simulink model "generic_src"  (Simulink 10.3)
settings: Solver=ode45  StartTime=0.0  StopTime=inf  RelTol=1e-3  EnableMultiTasking=on
undefined symbols (not defined in the file or in its folder): Area_Front, Area_Rear, ay_max_off, ay_max_on, ay_per_mu_max_off, ay_per_mu_max_on, Brake_ratio, brake_valve_ctrl_kP, cat1mode1_higher, cat1mode1_lower, cat1mode2_higher, cat1mode2_lower, cat1mode3_higher, cat1mode3_lower, cat2mode1_higher, cat2mode1_lower, cat2mode2_higher, cat2mode2_lower, cat2mode3_higher, cat2mode3_lower, delta_vel, diff_lock_fac, diff_lock_off, diff_lock_on, ESP_ctrl_kD, ESP_ctrl_kI, ESP_ctrl_kP, ESP_ctrl_restore_kI, ESP_min_throttle_fac, f_ax, f_slip, g, higherlimit_highvel, higherlimit_lowvel, highervel_fac, highervelocity_fac, InitialConditionForIntegrator, limit_acc, limit_selectlow, limit_starting, limit_vdiff, locktime_throttle, lowerlimit_highvel, lowerlimit_lowvel, lowervel_fac, lowervelocity_fac, min_throttle, MPS2KMPH, MSR_ctrl_kD, MSR_ctrl_kI, MSR_ctrl_kP, MSR_min_throttle_fac, PID_kP_sideslip, PID_kP_yawrate, RADpS2RpM, rBrake, RpM2RADpS, SH_SL_switch, sideslip_vel_corr, sidesplip_deviation_max ... (+35)
libraries: CarMaker4SL x136, simulink x55, simulink_extras x6
(part 3 of 9)

== system generic_src/CarMaker/IPG Vehicle/PowerTrain/PTControl Example/PTC MotorOut ==
  BusCreator : BusCreator  Inputs=12
  CreateBus PTC MotorOut0 : Subsystem
  CreateBus PTC MotorOut1 : Subsystem
  CreateBus PTC MotorOut10 : Subsystem
  CreateBus PTC MotorOut11 : Subsystem
  CreateBus PTC MotorOut2 : Subsystem
  CreateBus PTC MotorOut3 : Subsystem
  CreateBus PTC MotorOut4 : Subsystem
  CreateBus PTC MotorOut5 : Subsystem
  CreateBus PTC MotorOut6 : Subsystem
  CreateBus PTC MotorOut7 : Subsystem
  CreateBus PTC MotorOut8 : Subsystem
  CreateBus PTC MotorOut9 : Subsystem
  Ground PTC MotorOut{0..11} (12 alike) : Ground
  PTC MotorOut : Outport
  wires:
  CreateBus PTC MotorOut0/1(Out) -> BusCreator/1  "PTC MotorOut0"
  Ground PTC MotorOut0/1 -> CreateBus PTC MotorOut0/1(In)
  Ground PTC MotorOut3/1 -> CreateBus PTC MotorOut3/1(In)
  Ground PTC MotorOut1/1 -> CreateBus PTC MotorOut1/1(In)
  CreateBus PTC MotorOut1/1(Out) -> BusCreator/2  "PTC MotorOut1"
  Ground PTC MotorOut4/1 -> CreateBus PTC MotorOut4/1(In)
  Ground PTC MotorOut2/1 -> CreateBus PTC MotorOut2/1(In)
  CreateBus PTC MotorOut2/1(Out) -> BusCreator/3  "PTC MotorOut2"
  Ground PTC MotorOut5/1 -> CreateBus PTC MotorOut5/1(In)
  Ground PTC MotorOut6/1 -> CreateBus PTC MotorOut6/1(In)
  Ground PTC MotorOut7/1 -> CreateBus PTC MotorOut7/1(In)
  Ground PTC MotorOut8/1 -> CreateBus PTC MotorOut8/1(In)
  Ground PTC MotorOut9/1 -> CreateBus PTC MotorOut9/1(In)
  Ground PTC MotorOut10/1 -> CreateBus PTC MotorOut10/1(In)
  Ground PTC MotorOut11/1 -> CreateBus PTC MotorOut11/1(In)
  CreateBus PTC MotorOut4/1(Out) -> BusCreator/5  "PTC MotorOut4"
  CreateBus PTC MotorOut5/1(Out) -> BusCreator/6  "PTC MotorOut5"
  CreateBus PTC MotorOut6/1(Out) -> BusCreator/7  "PTC MotorOut6"
  CreateBus PTC MotorOut7/1(Out) -> BusCreator/8  "PTC MotorOut7"
  CreateBus PTC MotorOut8/1(Out) -> BusCreator/9  "PTC MotorOut8"
  CreateBus PTC MotorOut9/1(Out) -> BusCreator/10  "PTC MotorOut9"
  CreateBus PTC MotorOut10/1(Out) -> BusCreator/11  "PTC MotorOut10"
  CreateBus PTC MotorOut11/1(Out) -> BusCreator/12  "PTC MotorOut11"
  CreateBus PTC MotorOut3/1(Out) -> BusCreator/4  "PTC MotorOut3"
  BusCreator/1 -> PTC MotorOut/1  "CreateBus PTC MotorOut"

== system generic_src/CarMaker/IPG Vehicle/PowerTrain/PTControl Example/PTControl Example ==
  note: Minimalistic PTControl example model, that only works with
      | the 'Generic' powertrain and the 'Manual' gearbox.
  EngineIn : Inport
  VhclCtrl.PT : Inport  Port=2
  Bus Selector : BusSelector  OutputSignals=VhclCtrl Key,VhclCtrl Gas,VhclCtrl Clutch,VhclCtrl GearNo
  Bus Selector1 : BusSelector  OutputSignals=PTC EngineIn.PTC EngineIn Engine_on
  Engine : Subsystem
  ISG : Subsystem
  PTC : Subsystem
  PTC MiscOut : Outport  VectorParamsAs1DForOutWhenUnconnected=off
  EngineOut : Outport  Port=2  VectorParamsAs1DForOutWhenUnconnected=off
  ISGOut : Outport  Port=3  VectorParamsAs1DForOutWhenUnconnected=off
  ClutchOut Pos : Outport  Port=4  VectorParamsAs1DForOutWhenUnconnected=off
  GearBoxOut GearNoTrg : Outport  Port=5  VectorParamsAs1DForOutWhenUnconnected=off
  wires:
  VhclCtrl.PT/1 -> Bus Selector/1
  EngineIn/1 -> Bus Selector1/1
  Engine/1(EngineOut) -> EngineOut/1
  Bus Selector1/1 -> Engine/2(Engine_on), PTC/2(Engine_on)  "<PTC EngineIn Engine_on>"
  Bus Selector/2 -> Engine/1(Gas)  "<VhclCtrl Gas>"
  ISG/1(ISGOut) -> ISGOut/1
  PTC/1(PTC MiscOut) -> PTC MiscOut/1
  Bus Selector/4 -> GearBoxOut GearNoTrg/1  "<VhclCtrl GearNo>"
  Bus Selector/3 -> ClutchOut Pos/1  "<VhclCtrl Clutch>"
  Bus Selector/1 -> PTC/1(Key), ISG/1(Key)  "<VhclCtrl Key>"

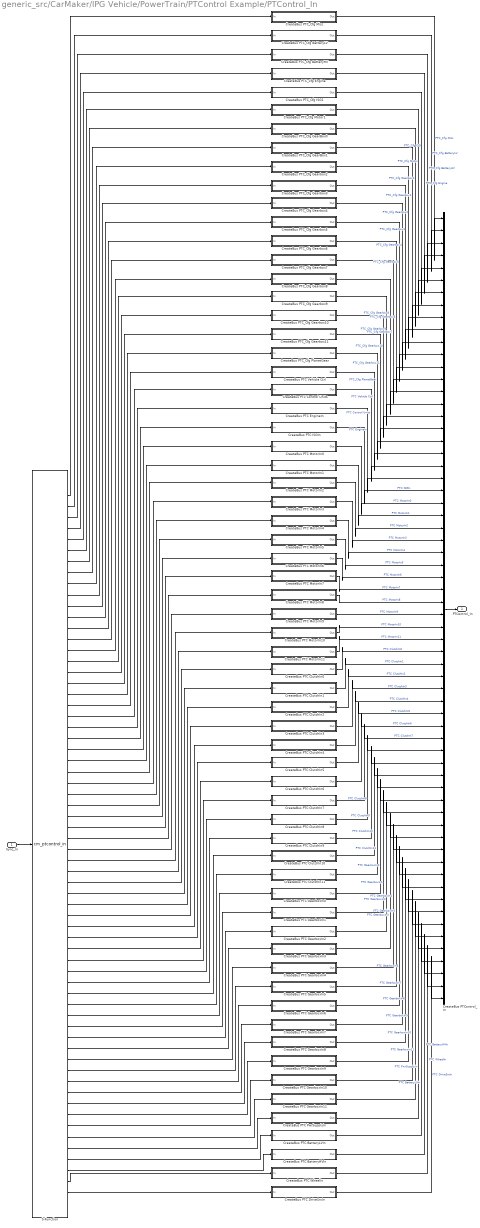
== system generic_src/CarMaker/IPG Vehicle/PowerTrain/PTControl Example/PTControl_In ==
  Sync_In : Inport
  CreateBus PTC BatteryHVIn : Subsystem
  CreateBus PTC BatteryLVIn : Subsystem
  CreateBus PTC ClutchIn0 : Subsystem
  CreateBus PTC ClutchIn1 : Subsystem
  CreateBus PTC ClutchIn10 : Subsystem
  CreateBus PTC ClutchIn11 : Subsystem
  CreateBus PTC ClutchIn2 : Subsystem
  CreateBus PTC ClutchIn3 : Subsystem
  CreateBus PTC ClutchIn4 : Subsystem
  CreateBus PTC ClutchIn5 : Subsystem
  CreateBus PTC ClutchIn6 : Subsystem
  CreateBus PTC ClutchIn7 : Subsystem
  CreateBus PTC ClutchIn8 : Subsystem
  CreateBus PTC ClutchIn9 : Subsystem
  CreateBus PTC Control Units : Subsystem
  CreateBus PTC DriveSrcIn : Subsystem
  CreateBus PTC EngineIn : Subsystem
  CreateBus PTC GearboxIn0 : Subsystem
  CreateBus PTC GearboxIn1 : Subsystem
  CreateBus PTC GearboxIn10 : Subsystem
  CreateBus PTC GearboxIn11 : Subsystem
  CreateBus PTC GearboxIn2 : Subsystem
  CreateBus PTC GearboxIn3 : Subsystem
  CreateBus PTC GearboxIn4 : Subsystem
  CreateBus PTC GearboxIn5 : Subsystem
  CreateBus PTC GearboxIn6 : Subsystem
  CreateBus PTC GearboxIn7 : Subsystem
  CreateBus PTC GearboxIn8 : Subsystem
  CreateBus PTC GearboxIn9 : Subsystem
  CreateBus PTC ISGIn : Subsystem
  CreateBus PTC MotorIn0 : Subsystem
  CreateBus PTC MotorIn1 : Subsystem
  CreateBus PTC MotorIn10 : Subsystem
  CreateBus PTC MotorIn11 : Subsystem
  CreateBus PTC MotorIn2 : Subsystem
  CreateBus PTC MotorIn3 : Subsystem
  CreateBus PTC MotorIn4 : Subsystem
  CreateBus PTC MotorIn5 : Subsystem
  CreateBus PTC MotorIn6 : Subsystem
  CreateBus PTC MotorIn7 : Subsystem
  CreateBus PTC MotorIn8 : Subsystem
  CreateBus PTC MotorIn9 : Subsystem
  CreateBus PTC PwrSupplyIn : Subsystem
  CreateBus PTC Vehicle Ctrl : Subsystem
  CreateBus PTC WheelIn : Subsystem
  CreateBus PTC_Cfg BatteryHV : Subsystem
  CreateBus PTC_Cfg BatteryLV : Subsystem
  CreateBus PTC_Cfg Engine : Subsystem
  CreateBus PTC_Cfg GearBox0 : Subsystem
  CreateBus PTC_Cfg GearBox1 : Subsystem
  CreateBus PTC_Cfg Gearbox10 : Subsystem
  CreateBus PTC_Cfg Gearbox11 : Subsystem
  CreateBus PTC_Cfg Gearbox2 : Subsystem
  CreateBus PTC_Cfg Gearbox3 : Subsystem
  CreateBus PTC_Cfg Gearbox4 : Subsystem
  CreateBus PTC_Cfg Gearbox5 : Subsystem
  CreateBus PTC_Cfg Gearbox6 : Subsystem
  CreateBus PTC_Cfg Gearbox7 : Subsystem
  CreateBus PTC_Cfg Gearbox8 : Subsystem
  CreateBus PTC_Cfg Gearbox9 : Subsystem
  CreateBus PTC_Cfg ISG1 : Subsystem
  CreateBus PTC_Cfg Misc : Subsystem
  CreateBus PTC_Cfg Motor1 : Subsystem
  CreateBus PTC_Cfg PlanetGear : Subsystem
  CreateBus PTControl_In : BusCreator  Inputs=64
  S-Function : S-Function  FunctionName=cm_ptcontrol_in  SFunctionDeploymentMode=off  EnableBusSupport=off
  PTControl_In : Outport  VectorParamsAs1DForOutWhenUnconnected=off
  wires:
  CreateBus PTControl_In/1 -> PTControl_In/1
  Sync_In/1 -> S-Function/1
  S-Function/2 -> CreateBus PTC_Cfg BatteryLV/1(In)
  CreateBus PTC_Cfg Misc/1(Out) -> CreateBus PTControl_In/1  "PTC_Cfg Misc"
  S-Function/1 -> CreateBus PTC_Cfg Misc/1(In)
  CreateBus PTC_Cfg Motor1/1(Out) -> CreateBus PTControl_In/6  "PTC_Cfg Motor"
  CreateBus PTC_Cfg Gearbox2/1(Out) -> CreateBus PTControl_In/9  "PTC_Cfg Gearbox2"
  S-Function/4 -> CreateBus PTC_Cfg Engine/1(In)
  S-Function/3 -> CreateBus PTC_Cfg BatteryHV/1(In)
  S-Function/7 -> CreateBus PTC_Cfg GearBox0/1(In)
  S-Function/14 -> CreateBus PTC_Cfg Gearbox7/1(In)
  S-Function/15 -> CreateBus PTC_Cfg Gearbox8/1(In)
  S-Function/17 -> CreateBus PTC_Cfg Gearbox10/1(In)
  S-Function/18 -> CreateBus PTC_Cfg Gearbox11/1(In)
  CreateBus PTC_Cfg GearBox1/1(Out) -> CreateBus PTControl_In/8  "PTC_Cfg Gearbox1"
  CreateBus PTC_Cfg Gearbox4/1(Out) -> CreateBus PTControl_In/11  "PTC_Cfg Gearbox4"
  CreateBus PTC_Cfg Gearbox5/1(Out) -> CreateBus PTControl_In/12  "PTC_Cfg Gearbox5"
  CreateBus PTC_Cfg Gearbox6/1(Out) -> CreateBus PTControl_In/13  "PTC_Cfg Gearbox6"
  CreateBus PTC_Cfg Gearbox7/1(Out) -> CreateBus PTControl_In/14  "PTC_Cfg Gearbox7"
  CreateBus PTC GearboxIn6/1(Out) -> CreateBus PTControl_In/54  "PTC GearboxIn6"
  CreateBus PTC ClutchIn6/1(Out) -> CreateBus PTControl_In/42  "PTC ClutchIn6"
  CreateBus PTC GearboxIn5/1(Out) -> CreateBus PTControl_In/53  "PTC GearboxIn5"
  CreateBus PTC GearboxIn9/1(Out) -> CreateBus PTControl_In/57  "PTC GearboxIn9"
  CreateBus PTC ClutchIn8/1(Out) -> CreateBus PTControl_In/44  "PTC ClutchIn8"
  S-Function/32 -> CreateBus PTC MotorIn8/1(In)
  CreateBus PTC MotorIn0/1(Out) -> CreateBus PTControl_In/24  "PTC MotorIn0"
  S-Function/8 -> CreateBus PTC_Cfg GearBox1/1(In)
  S-Function/46 -> CreateBus PTC ClutchIn10/1(In)
  S-Function/61 -> CreateBus PTC BatteryLVIn/1(In)
  S-Function/11 -> CreateBus PTC_Cfg Gearbox4/1(In)
  S-Function/37 -> CreateBus PTC ClutchIn1/1(In)
  S-Function/50 -> CreateBus PTC GearboxIn2/1(In)
  CreateBus PTC WheelIn/1(Out) -> CreateBus PTControl_In/63  "PTC WheelIn"
  S-Function/24 -> CreateBus PTC MotorIn0/1(In)
  CreateBus PTC_Cfg Gearbox3/1(Out) -> CreateBus PTControl_In/10  "PTC_Cfg Gearbox3"
  S-Function/51 -> CreateBus PTC GearboxIn3/1(In)
  S-Function/56 -> CreateBus PTC GearboxIn8/1(In)
  CreateBus PTC GearboxIn3/1(Out) -> CreateBus PTControl_In/51  "PTC GearboxIn3"
  CreateBus PTC MotorIn1/1(Out) -> CreateBus PTControl_In/25  "PTC MotorIn1"
  S-Function/10 -> CreateBus PTC_Cfg Gearbox3/1(In)
  CreateBus PTC DriveSrcIn/1(Out) -> CreateBus PTControl_In/64  "PTC DriveSrcIn"
  CreateBus PTC ISGIn/1(Out) -> CreateBus PTControl_In/23  "PTC ISGIn"
  CreateBus PTC ClutchIn11/1(Out) -> CreateBus PTControl_In/47  "PTC ClutchIn11"
  S-Function/20 -> CreateBus PTC Vehicle Ctrl/1(In)
  S-Function/47 -> CreateBus PTC ClutchIn11/1(In)
  S-Function/64 -> CreateBus PTC DriveSrcIn/1(In)
  CreateBus PTC ClutchIn10/1(Out) -> CreateBus PTControl_In/46  "PTC ClutchIn10"
  CreateBus PTC GearboxIn2/1(Out) -> CreateBus PTControl_In/50  "PTC GearboxIn2"
  CreateBus PTC GearboxIn0/1(Out) -> CreateBus PTControl_In/48  "PTC GearboxIn0"
  S-Function/16 -> CreateBus PTC_Cfg Gearbox9/1(In)
  S-Function/25 -> CreateBus PTC MotorIn1/1(In)
  S-Function/63 -> CreateBus PTC WheelIn/1(In)
  CreateBus PTC GearboxIn1/1(Out) -> CreateBus PTControl_In/49  "PTC GearboxIn1"
  S-Function/33 -> CreateBus PTC MotorIn9/1(In)
  CreateBus PTC BatteryLVIn/1(Out) -> CreateBus PTControl_In/61  "PTC BatteryLVIn"
  S-Function/58 -> CreateBus PTC GearboxIn10/1(In)
  S-Function/41 -> CreateBus PTC ClutchIn5/1(In)
  S-Function/5 -> CreateBus PTC_Cfg ISG1/1(In)
  S-Function/44 -> CreateBus PTC ClutchIn8/1(In)
  S-Function/45 -> CreateBus PTC ClutchIn9/1(In)
  CreateBus PTC GearboxIn11/1(Out) -> CreateBus PTControl_In/59  "PTC GearboxIn11"
  S-Function/9 -> CreateBus PTC_Cfg Gearbox2/1(In)
  S-Function/35 -> CreateBus PTC MotorIn11/1(In)
  S-Function/19 -> CreateBus PTC_Cfg PlanetGear/1(In)
  CreateBus PTC GearboxIn8/1(Out) -> CreateBus PTControl_In/56  "PTC GearboxIn8"
  S-Function/36 -> CreateBus PTC ClutchIn0/1(In)
  S-Function/53 -> CreateBus PTC GearboxIn5/1(In)
  CreateBus PTC GearboxIn10/1(Out) -> CreateBus PTControl_In/58  "PTC GearboxIn10"
  S-Function/6 -> CreateBus PTC_Cfg Motor1/1(In)
  CreateBus PTC PwrSupplyIn/1(Out) -> CreateBus PTControl_In/60  "PTC PwrSupplyIn"
  S-Function/43 -> CreateBus PTC ClutchIn7/1(In)
  CreateBus PTC_Cfg BatteryLV/1(Out) -> CreateBus PTControl_In/2  "PTC_Cfg BatteryLV"
  CreateBus PTC ClutchIn1/1(Out) -> CreateBus PTControl_In/37  "PTC ClutchIn1"
  S-Function/26 -> CreateBus PTC MotorIn2/1(In)
  CreateBus PTC_Cfg PlanetGear/1(Out) -> CreateBus PTControl_In/19  "PTC_Cfg PlanetGear"
  CreateBus PTC_Cfg Gearbox10/1(Out) -> CreateBus PTControl_In/17  "PTC_Cfg Gearbox10"
  CreateBus PTC ClutchIn7/1(Out) -> CreateBus PTControl_In/43  "PTC ClutchIn7"
  S-Function/54 -> CreateBus PTC GearboxIn6/1(In)
  S-Function/29 -> CreateBus PTC MotorIn5/1(In)
  CreateBus PTC_Cfg BatteryHV/1(Out) -> CreateBus PTControl_In/3  "PTC_Cfg BatteryHV"
  S-Function/13 -> CreateBus PTC_Cfg Gearbox6/1(In)
  CreateBus PTC ClutchIn9/1(Out) -> CreateBus PTControl_In/45  "PTC ClutchIn9"
  CreateBus PTC GearboxIn4/1(Out) -> CreateBus PTControl_In/52  "PTC GearboxIn4"
  S-Function/57 -> CreateBus PTC GearboxIn9/1(In)
  CreateBus PTC GearboxIn7/1(Out) -> CreateBus PTControl_In/55  "PTC GearboxIn7"
  S-Function/60 -> CreateBus PTC PwrSupplyIn/1(In)
  CreateBus PTC BatteryHVIn/1(Out) -> CreateBus PTControl_In/62  "PTC BatteryHVIn"
  S-Function/49 -> CreateBus PTC GearboxIn1/1(In)
  S-Function/55 -> CreateBus PTC GearboxIn7/1(In)
  S-Function/21 -> CreateBus PTC Control Units/1(In)
  CreateBus PTC ClutchIn5/1(Out) -> CreateBus PTControl_In/41  "PTC ClutchIn5"
  CreateBus PTC ClutchIn4/1(Out) -> CreateBus PTControl_In/40  "PTC ClutchIn4"
  S-Function/38 -> CreateBus PTC ClutchIn2/1(In)
  CreateBus PTC Control Units/1(Out) -> CreateBus PTControl_In/21  "PTC Control Units"
  S-Function/40 -> CreateBus PTC ClutchIn4/1(In)
  CreateBus PTC MotorIn11/1(Out) -> CreateBus PTControl_In/35  "PTC MotorIn11"
  CreateBus PTC ClutchIn3/1(Out) -> CreateBus PTControl_In/39  "PTC ClutchIn3"
  S-Function/39 -> CreateBus PTC ClutchIn3/1(In)
  CreateBus PTC MotorIn2/1(Out) -> CreateBus PTControl_In/26  "PTC MotorIn2"
  CreateBus PTC ClutchIn2/1(Out) -> CreateBus PTControl_In/38  "PTC ClutchIn2"
  CreateBus PTC_Cfg ISG1/1(Out) -> CreateBus PTControl_In/5  "PTC_Cfg ISG"
  CreateBus PTC ClutchIn0/1(Out) -> CreateBus PTControl_In/36  "PTC ClutchIn0"
  S-Function/52 -> CreateBus PTC GearboxIn4/1(In)
  CreateBus PTC EngineIn/1(Out) -> CreateBus PTControl_In/22  "PTC EngineIn"
  CreateBus PTC_Cfg GearBox0/1(Out) -> CreateBus PTControl_In/7  "PTC_Cfg Gearbox0"
  S-Function/42 -> CreateBus PTC ClutchIn6/1(In)
  S-Function/34 -> CreateBus PTC MotorIn10/1(In)
  CreateBus PTC MotorIn9/1(Out) -> CreateBus PTControl_In/33  "PTC MotorIn9"
  S-Function/30 -> CreateBus PTC MotorIn6/1(In)
  S-Function/12 -> CreateBus PTC_Cfg Gearbox5/1(In)
  CreateBus PTC MotorIn8/1(Out) -> CreateBus PTControl_In/32  "PTC MotorIn8"
  CreateBus PTC MotorIn7/1(Out) -> CreateBus PTControl_In/31  "PTC MotorIn7"
  S-Function/31 -> CreateBus PTC MotorIn7/1(In)
  CreateBus PTC MotorIn6/1(Out) -> CreateBus PTControl_In/30  "PTC MotorIn6"
  CreateBus PTC MotorIn4/1(Out) -> CreateBus PTControl_In/28  "PTC MotorIn4"
  S-Function/62 -> CreateBus PTC BatteryHVIn/1(In)
  S-Function/27 -> CreateBus PTC MotorIn3/1(In)
  S-Function/28 -> CreateBus PTC MotorIn4/1(In)
  CreateBus PTC MotorIn5/1(Out) -> CreateBus PTControl_In/29  "PTC MotorIn5"
  CreateBus PTC MotorIn3/1(Out) -> CreateBus PTControl_In/27  "PTC MotorIn3"
  S-Function/23 -> CreateBus PTC ISGIn/1(In)
  S-Function/22 -> CreateBus PTC EngineIn/1(In)
  CreateBus PTC_Cfg Engine/1(Out) -> CreateBus PTControl_In/4  "PTC_Cfg Engine"
  S-Function/48 -> CreateBus PTC GearboxIn0/1(In)
  S-Function/59 -> CreateBus PTC GearboxIn11/1(In)
  CreateBus PTC Vehicle Ctrl/1(Out) -> CreateBus PTControl_In/20  "PTC Vehicle Ctrl"
  CreateBus PTC MotorIn10/1(Out) -> CreateBus PTControl_In/34  "PTC MotorIn10"
  CreateBus PTC_Cfg Gearbox11/1(Out) -> CreateBus PTControl_In/18  "PTC_Cfg Gearbox11"
  CreateBus PTC_Cfg Gearbox9/1(Out) -> CreateBus PTControl_In/16  "PTC_Cfg Gearbox9"
  CreateBus PTC_Cfg Gearbox8/1(Out) -> CreateBus PTControl_In/15  "PTC_Cfg Gearbox8"

== system generic_src/CarMaker/IPG Vehicle/PowerTrain/PTControl Example/PTControl_Out ==
  PTC MiscOut : Inport
  PTC EngineOut : Inport  Port=2
  PTC ISGOut : Inport  Port=3
  PTC MotorOut : Inport  Port=4
  PTC ClutchOut : Inport  Port=5
  PTC GearboxOut : Inport  Port=6
  PTC PwrSupplyOut : Inport  Port=7
  PTC BattLV_Out : Inport  Port=8
  PTC BattHV_Out : Inport  Port=9
  PTC WheelOut : Inport  Port=10
  Bus Selector1 : BusSelector  OutputSignals=PTC MotorOut0,PTC MotorOut1,PTC MotorOut2,PTC MotorOut3,PTC MotorOut4,PTC MotorOut5,PTC MotorOut6,PTC MotorOut7,PTC MotorOut8,PTC MotorOut9,PTC MotorOut10,PTC MotorOut11
  Bus Selector2 : BusSelector  OutputSignals=PTC ClutchOut0,PTC ClutchOut1,PTC ClutchOut2,PTC ClutchOut3,PTC ClutchOut4,PTC ClutchOut5,PTC ClutchOut6,PTC ClutchOut7,PTC ClutchOut8,PTC ClutchOut9,PTC ClutchOut10,PTC ClutchOut11
  Bus Selector3 : BusSelector  OutputSignals=PTC GearBoxOut0,PTC GearBoxOut1,PTC GearBoxOut2,PTC GearBoxOut3,PTC GearBoxOut4,PTC GearBoxOut5,PTC GearBoxOut6,PTC GearBoxOut7,PTC GearBoxOut8,PTC GearBoxOut9,PTC GearBoxOut10,PTC GearBoxOut11
  PTControl_Out : S-Function  FunctionName=cm_ptcontrol_out  SFunctionDeploymentMode=off  EnableBusSupport=off
  wires:
  PTC MotorOut/1 -> Bus Selector1/1
  PTC ISGOut/1 -> PTControl_Out/3
  PTC EngineOut/1 -> PTControl_Out/2
  PTC MiscOut/1 -> PTControl_Out/1
  Bus Selector1/1 -> PTControl_Out/4  "<PTC MotorOut0>"
  Bus Selector1/2 -> PTControl_Out/5  "<PTC MotorOut1>"
  Bus Selector1/3 -> PTControl_Out/6  "<PTC MotorOut2>"
  Bus Selector1/4 -> PTControl_Out/7  "<PTC MotorOut3>"
  Bus Selector1/5 -> PTControl_Out/8  "<PTC MotorOut4>"
  Bus Selector1/6 -> PTControl_Out/9  "<PTC MotorOut5>"
  Bus Selector1/7 -> PTControl_Out/10  "<PTC MotorOut6>"
  Bus Selector1/8 -> PTControl_Out/11  "<PTC MotorOut7>"
  Bus Selector1/9 -> PTControl_Out/12  "<PTC MotorOut8>"
  Bus Selector1/10 -> PTControl_Out/13  "<PTC MotorOut9>"
  Bus Selector1/11 -> PTControl_Out/14  "<PTC MotorOut10>"
  Bus Selector1/12 -> PTControl_Out/15  "<PTC MotorOut11>"
  PTC ClutchOut/1 -> Bus Selector2/1
  Bus Selector2/1 -> PTControl_Out/16  "<PTC ClutchOut0>"
  Bus Selector2/2 -> PTControl_Out/17  "<PTC ClutchOut1>"
  Bus Selector2/3 -> PTControl_Out/18  "<PTC ClutchOut2>"
  Bus Selector2/4 -> PTControl_Out/19  "<PTC ClutchOut3>"
  Bus Selector2/5 -> PTControl_Out/20  "<PTC ClutchOut4>"
  Bus Selector2/6 -> PTControl_Out/21  "<PTC ClutchOut5>"
  Bus Selector2/7 -> PTControl_Out/22  "<PTC ClutchOut6>"
  Bus Selector2/8 -> PTControl_Out/23  "<PTC ClutchOut7>"
  Bus Selector2/9 -> PTControl_Out/24  "<PTC ClutchOut8>"
  Bus Selector2/10 -> PTControl_Out/25  "<PTC ClutchOut9>"
  Bus Selector2/11 -> PTControl_Out/26  "<PTC ClutchOut10>"
  Bus Selector2/12 -> PTControl_Out/27  "<PTC ClutchOut11>"
  PTC GearboxOut/1 -> Bus Selector3/1
  Bus Selector3/1 -> PTControl_Out/28  "<PTC GearBoxOut0>"
  Bus Selector3/2 -> PTControl_Out/29  "<PTC GearBoxOut1>"
  Bus Selector3/3 -> PTControl_Out/30  "<PTC GearBoxOut2>"
  Bus Selector3/4 -> PTControl_Out/31  "<PTC GearBoxOut3>"
  Bus Selector3/5 -> PTControl_Out/32  "<PTC GearBoxOut4>"
  Bus Selector3/6 -> PTControl_Out/33  "<PTC GearBoxOut5>"
  Bus Selector3/7 -> PTControl_Out/34  "<PTC GearBoxOut6>"
  Bus Selector3/8 -> PTControl_Out/35  "<PTC GearBoxOut7>"
  Bus Selector3/9 -> PTControl_Out/36  "<PTC GearBoxOut8>"
  Bus Selector3/10 -> PTControl_Out/37  "<PTC GearBoxOut9>"
  Bus Selector3/11 -> PTControl_Out/38  "<PTC GearBoxOut10>"
  Bus Selector3/12 -> PTControl_Out/39  "<PTC GearBoxOut11>"
  PTC PwrSupplyOut/1 -> PTControl_Out/40
  PTC BattLV_Out/1 -> PTControl_Out/41
  PTC BattHV_Out/1 -> PTControl_Out/42
  PTC WheelOut/1 -> PTControl_Out/43

== system generic_src/CarMaker/IPG Vehicle/Brake/HydBrakeCU Example/ESP Controller/ESP General System ==
  ESP Input Signals : Inport
  User Input Signals : Inport  Port=2
  Vehicle Input Params : Inport  Port=3
  Ideal_In : Inport  Port=4
  ABS : Subsystem
  ASR : Subsystem
  Bus Creator : BusCreator  Inputs=7
  Bus Creator2 : BusCreator  Inputs=5
  Bus Creator3 : BusCreator  Inputs=6
  Bus Creator4 : BusCreator  Inputs=4
  ESP : Subsystem
  HSA : Subsystem
  Master Controller : Subsystem
  Signal Handling : Subsystem
  ESP Out : Outport  VectorParamsAs1DForOutWhenUnconnected=off
  wires:
  Bus Creator/1 -> ESP Out/1
  ESP Input Signals/1 -> Signal Handling/1(ESP In)
  ESP/1(ESP On) -> Master Controller/2(ESP On)  "ESP On"
  ESP/2(Pilot Valves) -> Bus Creator2/1  "Pilot Valves"
  ESP/3(Suction Valves) -> Bus Creator2/2  "Suction Valves"
  ESP/4(Brake Valves) -> Bus Creator2/3  "Brake Valves"
  ESP/5(Pump Ctrl) -> Bus Creator2/4  "Pump Ctrl"
  ESP/6(Gas_Out) -> Bus Creator2/5  "Gas_Out"
  Bus Creator2/1 -> Master Controller/3(ESP Bus)  "ESP Bus"
  ASR/1(ASR On) -> Master Controller/4(ASR On)  "ASR On"
  ABS/1(ABS On) -> Master Controller/6(ABS On)  "ABS On"
  Bus Creator3/1 -> Master Controller/5(ASR Bus)  "ASR Bus"
  Master Controller/1(ECU Flags) -> Bus Creator/1  "ECU Flags"
  Master Controller/2(Brake Valves) -> Bus Creator/2  "Brake Valves"
  Master Controller/3(Pilot Valves) -> Bus Creator/3  "Pilot Valves"
  Master Controller/4(Suction Valves) -> Bus Creator/4  "Suction Valves"
  Master Controller/5(Pump Ctrl) -> Bus Creator/5  "Pump Ctrl"
  ASR/2(Pilot Valves) -> Bus Creator3/1  "Pilot Valves"
  ASR/3(Suction Valves) -> Bus Creator3/2  "Suction Valves"
  ASR/4(Brake Valves) -> Bus Creator3/3  "Brake Valves"
  ASR/5(Pump Ctrl) -> Bus Creator3/4  "Pump Ctrl"
  ASR/6(Gas_out) -> Bus Creator3/5  "Gas_Out"
  ABS/2(Pilot Valves) -> Bus Creator4/1  "Pilot Valves"
  ABS/3(Suction Valves) -> Bus Creator4/2  "Suction Valves"
  ABS/4(Brake Valves) -> Bus Creator4/3  "Brake Valves"
  ABS/5(Pump Ctrl) -> Bus Creator4/4  "Pump Ctrl"
  Bus Creator4/1 -> Master Controller/7(ABS Bus)  "ABS Bus"
  User Input Signals/1 -> Master Controller/10(User In), ESP/4(User_In), ASR/4(User_In), ABS/4(User_In)
  Vehicle Input Params/1 -> Signal Handling/2(Vehicle Params), ESP/3(Vehicle Params), ASR/3(Vehicle Params), ABS/3(Vehicle Params)
  ASR/7(Diff_Torque) -> Bus Creator3/6  "Diff_Torque"
  Master Controller/6(Diff_Torque) -> Bus Creator/6  "Diff_Torque"
  Ideal_In/1 -> HSA/2(Ideal_In), ABS/2(Ideal_In), ESP/2(Ideal_In), ASR/2(Ideal_In)
  Master Controller/7(VC_Out) -> Bus Creator/7  "VC_Out"
  Signal Handling/2(Signal Bus ESP) -> ESP/1(ESP Signal Bus)
  Signal Handling/3(Signal Bus ASR) -> ASR/1(ASR Signal Bus)
  Signal Handling/4(Signal Bus ABS) -> ABS/1(ABS Signal Bus)
  Signal Handling/5(Signal Bus HSA) -> HSA/1(HSA Signal Bus)
  HSA/1(HSA On) -> Master Controller/8(HSA On)
  HSA/2(BrakePark_Out) -> Master Controller/9(HSA Bus)  "BrakePark"
  Signal Handling/1(Signal Bus Master Controller) -> Master Controller/1(Signal In)

== system generic_src/CarMaker/IPG Vehicle/Brake/HydBrakeCU Example/ESP Controller/ESP Input Signals ==
  HydBrakeCtrl_In : Inport
  " " : simulink_extras/Transformations/Radians to Degrees
  "   " : simulink_extras/Transformations/Radians to Degrees
  Bus Creator1 : BusCreator  Inputs=20
  Bus Selector : BusSelector  OutputSignals=Omega_B z,Acc_B y,Acc_B x
  Bus Selector1 : BusSelector  OutputSignals=HydBrakeCU pMC,HydBrakeCU pWB_FL,HydBrakeCU pWB_FR,HydBrakeCU pWB_RL,HydBrakeCU pWB_RR,HydBrakeCU Park,HydBrakeCU Pedal
  Car InertialSensor : CarMaker4SL/Sensors/Inertial Sensor  xname=Vhcl.YRS  xstime=Continuous
      settings: SourceProductName=CarMaker4SL
  Gain{,6,9..10,12..17} (10 alike) : Gain  SaturateOnIntegerOverflow=on  OutDataTypeStr=Inherit: Same as input  ParamDataTypeStr=Inherit: Same as input
  Gain{1..5,11} (6 alike) : Gain  Gain=RADpS2RpM  SaturateOnIntegerOverflow=on  OutDataTypeStr=Inherit: Same as input  ParamDataTypeStr=Inherit: Same as input
  Gain7 : Gain  Gain=1/g  SaturateOnIntegerOverflow=on  OutDataTypeStr=Inherit: Same as input  ParamDataTypeStr=Inherit: Same as input
  Gain8 : Gain  Gain=1/g  SaturateOnIntegerOverflow=on  OutDataTypeStr=Inherit: Same as input  ParamDataTypeStr=Inherit: Same as input
  Read CM Dict1 : CarMaker4SL/Read CM Dict  xname=Car.WheelSpd_FL  xsync=off  xstime=Continuous
  Read CM Dict10 : CarMaker4SL/Read CM Dict  xname=PT.Clutch.0.rotv_out  xsync=off  xstime=Continuous
  Read CM Dict11 : CarMaker4SL/Read CM Dict  xname=Steer.WhlAng  xsync=off  xstime=Continuous
  Read CM Dict12 : CarMaker4SL/Read CM Dict  xname=PT.Engine.Trq  xsync=off  xstime=Continuous
  Read CM Dict15 : CarMaker4SL/Read CM Dict  xname=PT.GearBox.0.GearNo  xsync=off  xstime=Continuous
  Read CM Dict2 : CarMaker4SL/Read CM Dict  xname=Car.WheelSpd_FR  xsync=off  xstime=Continuous
  Read CM Dict3 : CarMaker4SL/Read CM Dict  xname=Car.WheelSpd_RL  xsync=off  xstime=Continuous
  Read CM Dict4 : CarMaker4SL/Read CM Dict  xname=Car.WheelSpd_RR  xsync=off  xstime=Continuous
  Read CM Dict7 : CarMaker4SL/Read CM Dict  xname=PT.Engine.rotv  xsync=off  xstime=Continuous
  Read CM Dict9 : CarMaker4SL/Read CM Dict  xname=VC.Gas  xsync=off  xstime=Continuous
  Terminator : Terminator
  ESP Signals : Outport  VectorParamsAs1DForOutWhenUnconnected=off
  wires:
  Gain9/1 -> Bus Creator1/9  "Engine crankshaft output torque [Nm]"
  Gain13/1 -> Bus Creator1/14  "GearState [-]"
  " "/1 -> Bus Creator1/13  "Steering Wheel Angle [deg]"
  Gain11/1 -> Bus Creator1/12  "Torque Converter Speed [rpm]"
  Gain10/1 -> Bus Creator1/10  "Master Cylinder Pressure [bar]"
  Gain8/1 -> Bus Creator1/7  "Sensor Longitudinal acceleration [g]"
  Gain7/1 -> Bus Creator1/6  "Sensor Lateral acceleration [g]"
  "   "/1 -> Bus Creator1/5  "Sensor YawRate [degs]"
  Gain4/1 -> Bus Creator1/4  "WheelSpd RR [rpm]"
  Gain5/1 -> Bus Creator1/3  "WheelSpd RL [rpm]"
  Gain3/1 -> Bus Creator1/2  "WheelSpd FR [rpm]"
  Gain2/1 -> Bus Creator1/1  "WheelSpd FL [rpm]"
  Read CM Dict15/1 -> Gain13/1  "GearNumber [-]"
  Gain1/1 -> Bus Creator1/8  "Engine Speed [rpm]"
  Bus Selector/1 -> "   "/1  "<Omega_B z>"
  Bus Selector/3 -> Gain8/1  "<Acc_B x>"
  Car InertialSensor/2 -> Bus Selector/1
  Read CM Dict11/1 -> " "/1  "Steering Angle [rad]"
  Read CM Dict10/1 -> Gain11/1  "Clucth OutShaft [rad/s]"
  Read CM Dict9/1 -> Gain/1  "Accelerator pedal [-]"
  Bus Selector1/1 -> Gain10/1  "<HydBrakeCU pMC>"
  Read CM Dict1/1 -> Gain2/1  "WheelSpd FL [rad]/s]"
  Read CM Dict2/1 -> Gain3/1  "WheelSpd FR [rad/s]"
  Read CM Dict3/1 -> Gain5/1  "WheelSpd RL [rad/s]"
  Bus Selector/2 -> Gain7/1  "<Acc_B y>"
  Read CM Dict4/1 -> Gain4/1  "WheelSpd RR [rad/s]"
  Gain/1 -> Bus Creator1/11  "Throttle Valve Position"
  Read CM Dict12/1 -> Gain9/1  "Engine Torque [Nm]"
  Read CM Dict7/1 -> Gain1/1  "Engine RotVel [rad/s]"
  Bus Creator1/1 -> ESP Signals/1
  Bus Selector1/5 -> Gain15/1  "<HydBrakeCU pWB_RR>"
  Bus Selector1/4 -> Gain14/1  "<HydBrakeCU pWB_RL>"
  Bus Selector1/3 -> Gain12/1  "<HydBrakeCU pWB_FR>"
  Bus Selector1/2 -> Gain6/1  "<HydBrakeCU pWB_FL>"
  Gain6/1 -> Bus Creator1/15  "Cylinder Pressure FL [bar]"
  Gain12/1 -> Bus Creator1/16  "Cylinder Pressure FR [bar]"
  Gain14/1 -> Bus Creator1/17  "Cylinder Pressure RL [bar]"
  Gain15/1 -> Bus Creator1/18  "Cylinder Pressure RR [bar]"
  HydBrakeCtrl_In/1 -> Bus Selector1/1
  Car InertialSensor/1 -> Terminator/1
  Bus Selector1/6 -> Gain16/1  "<HydBrakeCU Park>"
  Gain16/1 -> Bus Creator1/19  "Park Brake Position"
  Bus Selector1/7 -> Gain17/1  "<HydBrakeCU Pedal>"
  Gain17/1 -> Bus Creator1/20  "Brake Pedal Position"

== system generic_src/CarMaker/IPG Vehicle/Brake/HydBrakeCU Example/ESP Controller/Ideal Input Signals ==
  Bus Creator1 : BusCreator  Inputs=8
  Bus Creator2 : BusCreator  Inputs=4
  Bus Creator3 : BusCreator  Inputs=2
  Bus Creator4 : BusCreator  Inputs=2
  Bus Creator5 : BusCreator  Inputs=3
  Bus Creator6 : BusCreator  Inputs=2
  Read CM Dict1 : CarMaker4SL/Read CM Dict  xname=Car.Pitch  xsync=off  xstime=Continuous
  Read CM Dict10 : CarMaker4SL/Read CM Dict  xname=Car.FzRL  xsync=off  xstime=Continuous
  Read CM Dict11 : CarMaker4SL/Read CM Dict  xname=Car.YawRate  xsync=off  xstime=Continuous
  Read CM Dict13 : CarMaker4SL/Read CM Dict  xname=Car.CRL.Trq_T2W  xsync=off  xstime=Continuous
  Read CM Dict14 : CarMaker4SL/Read CM Dict  xname=Car.LongSlipRL  xsync=off  xstime=Continuous
  Read CM Dict16 : CarMaker4SL/Read CM Dict  xname=Car.CRR.Trq_T2W  xsync=off  xstime=Continuous
  Read CM Dict17 : CarMaker4SL/Read CM Dict  xname=Car.FzRR  xsync=off  xstime=Continuous
  Read CM Dict19 : CarMaker4SL/Read CM Dict  xname=Car.LongSlipRR  xsync=off  xstime=Continuous
  Read CM Dict2 : CarMaker4SL/Read CM Dict  xname=Car.v  xsync=off  xstime=Continuous
  Read CM Dict3 : CarMaker4SL/Read CM Dict  xname=Car.muRoadFR  xsync=off  xstime=Continuous
  Read CM Dict4 : CarMaker4SL/Read CM Dict  xname=Car.muRoadRL  xsync=off  xstime=Continuous
  Read CM Dict5 : CarMaker4SL/Read CM Dict  xname=Car.SideSlipAngle  xsync=off  xstime=Continuous
  Read CM Dict6 : CarMaker4SL/Read CM Dict  xname=Car.muRoadFL  xsync=off  xstime=Continuous
  Read CM Dict7 : CarMaker4SL/Read CM Dict  xname=Car.muRoadRR  xsync=off  xstime=Continuous
  Read CM Dict8 : CarMaker4SL/Read CM Dict  xname=Car.vx  xsync=off  xstime=Continuous
  Read CM Dict9 : CarMaker4SL/Read CM Dict  xname=Car.vy  xsync=off  xstime=Continuous
  Ideal_In : Outport  VectorParamsAs1DForOutWhenUnconnected=off
  wires:
  Read CM Dict17/1 -> Bus Creator4/2  "Ideal_FzRR"
  Read CM Dict10/1 -> Bus Creator4/1  "Ideal_FzRL"
  Read CM Dict16/1 -> Bus Creator3/2  "Ideal_Trq2WRR"
  Read CM Dict13/1 -> Bus Creator3/1  "Ideal_Trq2WRL"
  Read CM Dict6/1 -> Bus Creator2/1  "Ideal_muFL"
  Read CM Dict3/1 -> Bus Creator2/2  "Ideal_muFR"
  Read CM Dict4/1 -> Bus Creator2/3  "Ideal_muRL"
  Read CM Dict7/1 -> Bus Creator2/4  "Ideal_muRR"
  Bus Creator1/1 -> Ideal_In/1
  Read CM Dict1/1 -> Bus Creator1/1  "Ideal_Pitch"
  Read CM Dict5/1 -> Bus Creator1/3  "Ideal_SideSlipAngle"
  Read CM Dict2/1 -> Bus Creator5/1  "Ideal_Velocity"
  Read CM Dict8/1 -> Bus Creator5/2  "Ideal_Velocity_x"
  Bus Creator5/1 -> Bus Creator1/2  "Ideal_Velocity"
  Read CM Dict9/1 -> Bus Creator5/3  "Ideal_Velocity_y"
  Read CM Dict14/1 -> Bus Creator6/1  "Ideal_SlipRL"
  Read CM Dict19/1 -> Bus Creator6/2  "Ideal_SlipRR"
  Read CM Dict11/1 -> Bus Creator1/4  "Ideal_YawRate"
  Bus Creator2/1 -> Bus Creator1/5  "Ideal_mu"
  Bus Creator3/1 -> Bus Creator1/6  "Idea_Trq2W"
  Bus Creator4/1 -> Bus Creator1/7  "Ideal_Fz"
  Bus Creator6/1 -> Bus Creator1/8  "Ideal_Slip"

== system generic_src/CarMaker/IPG Vehicle/Brake/HydBrakeCU Example/ESP Controller/Output Signals ESP ==
  ESP Out : Inport
  Bus Creator : BusCreator  Inputs=6
  Bus Selector : BusSelector  OutputSignals=ECU Flags,Brake Valves,Pilot Valves,Suction Valves,Pump Ctrl,VC_Out.BrakePark,VC_Out.Brake Pedal Position,Diff_Torque,VC_Out.Load_lim
  Bus Selector1 : BusSelector  OutputSignals=ESP On,ASR On,ABS On,HSA On
  Bus Selector2 : BusSelector  OutputSignals=ASR On,MSR On,BMR On
  Bus Selector4 : BusSelector  OutputSignals=FrontDiff_Torque
  Data Type Conversion : DataTypeConversion
  Define CM Dict1 : CarMaker4SL/Define CM Dict  xname=ESP.ASR.MSR.active  xmono=off  xtype=Char  xdvaplace=VC  xnstates=2  xfirststate=0  xinitial=0
  Define CM Dict10 : CarMaker4SL/Define CM Dict  xname=ESP.ESP.active  xmono=off  xtype=Char  xdvaplace=VC  xnstates=2  xfirststate=0  xinitial=0
  Define CM Dict2 : CarMaker4SL/Define CM Dict  xname=ESP.ASR.BMR.active  xmono=off  xtype=Char  xdvaplace=VC  xnstates=2  xfirststate=0  xinitial=0
  Define CM Dict3 : CarMaker4SL/Define CM Dict  xname=ESP.ASR.active  xmono=off  xtype=Char  xdvaplace=VC  xnstates=2  xfirststate=0  xinitial=0
  Define CM Dict4 : CarMaker4SL/Define CM Dict  xname=ESP.HSA.active  xmono=off  xtype=Char  xdvaplace=VC  xnstates=2  xfirststate=0  xinitial=0
  Define CM Dict6 : CarMaker4SL/Define CM Dict  xname=ESP.ESP.lamp  xmono=off  xtype=Char  xdvaplace=VC  xnstates=2  xfirststate=0  xinitial=0
  Define CM Dict9 : CarMaker4SL/Define CM Dict  xname=ESP.ABS.Active  xmono=off  xtype=Char  xdvaplace=VC  xnstates=2  xfirststate=0  xinitial=0
  Logical Operator : Logic  Operator=OR  AllPortsSameDT=off  OutDataTypeStr=boolean
  Read CM Dict3 : CarMaker4SL/Read CM Dict  xname=ESP.User.ESP_off  xsync=off  xstime=Continuous
  Write CM Dict : CarMaker4SL/Write CM Dict  xname=PT.ECU.Load_lim_max  xsync=off
  Write CM Dict12 : CarMaker4SL/Write CM Dict  xname=ESP.ASR.MSR.active  xsync=off
  Write CM Dict13 : CarMaker4SL/Write CM Dict  xname=ESP.ASR.BMR.active  xsync=off
  Write CM Dict15 : CarMaker4SL/Write CM Dict  xname=ESP.ASR.active  xsync=off
  Write CM Dict17 : CarMaker4SL/Write CM Dict  xname=ESP.ABS.Active  xsync=off
  Write CM Dict18 : CarMaker4SL/Write CM Dict  xname=ESP.ESP.active  xsync=off
  Write CM Dict19 : CarMaker4SL/Write CM Dict  xname=PT.Gen.DL.FDiff.DVA.Trq_A2B  xsync=off
  Write CM Dict20 : CarMaker4SL/Write CM Dict  xname=ESP.HSA.active  xsync=off
  Write CM Dict21 : CarMaker4SL/Write CM Dict  xname=ESP.ESP.lamp  xsync=off
  HydBrakeCU_Out : Outport  VectorParamsAs1DForOutWhenUnconnected=off
  wires:
  ESP Out/1 -> Bus Selector/1
  Bus Selector/1 -> Bus Selector1/1  "<ECU Flags>"
  Bus Selector1/2 -> Bus Selector2/1  "<ASR On>"
  Bus Selector1/1 -> Logical Operator/2, Write CM Dict18/1  "<ESP On>"
  Bus Selector1/3 -> Write CM Dict17/1  "<ABS On>"
  Bus Selector2/1 -> Write CM Dict15/1  "<ASR On>"
  Bus Selector2/2 -> Write CM Dict12/1  "<MSR On>"
  Bus Selector2/3 -> Write CM Dict13/1  "<BMR On>"
  Bus Selector4/1 -> Write CM Dict19/1  "<FrontDiff_Torque>"
  Bus Selector/8 -> Bus Selector4/1  "<Diff_Torque>"
  Bus Selector1/4 -> Write CM Dict20/1  "<HSA On>"
  Logical Operator/1 -> Data Type Conversion/1
  Read CM Dict3/1 -> Logical Operator/1
  Data Type Conversion/1 -> Write CM Dict21/1
  Bus Selector/2 -> Bus Creator/1  "<Brake Valves>"
  Bus Selector/3 -> Bus Creator/2  "<Pilot Valves>"
  Bus Selector/4 -> Bus Creator/3  "<Suction Valves>"
  Bus Selector/5 -> Bus Creator/4  "<Pump Ctrl>"
  Bus Creator/1 -> HydBrakeCU_Out/1
  Bus Selector/6 -> Bus Creator/5  "<BrakePark>"
  Bus Selector/9 -> Write CM Dict/1  "<Load_lim>"
  Bus Selector/7 -> Bus Creator/6  "<Brake Pedal Position>"

== system generic_src/CarMaker/IPG Vehicle/Brake/HydBrakeCU Example/ESP Controller/User Input Signals1 ==
  note: User_Drive: 1 = Front; 2 = Rear; 3 = AllWheel
  Bus Creator1 : BusCreator  Inputs=5
  Bus Creator2 : BusCreator  Inputs=5
  Bus Creator3 : BusCreator  Inputs=2
  Bus Creator4 : BusCreator  Inputs=2
  Define CM Dict1 : CarMaker4SL/Define CM Dict  xname=ESP.User.ESP_off  xmono=off  xtype=Char  xdvaplace=IO_Out  xnstates=2  xfirststate=0  xinitial=0
  Define CM Dict10 : CarMaker4SL/Define CM Dict  xname=ESP.User.HSA_off  xmono=off  xtype=Char  xdvaplace=IO_Out  xnstates=2  xfirststate=0  xinitial=0
  Define CM Dict11 : CarMaker4SL/Define CM Dict  xname=ESP.User.oneWheel_on  xmono=off  xtype=Char  xdvaplace=IO_Out  xnstates=2  xfirststate=0  xinitial=0
  Define CM Dict2 : CarMaker4SL/Define CM Dict  xname=ESP.User.ASR_off  xmono=off  xtype=Char  xdvaplace=IO_Out  xnstates=2  xfirststate=0  xinitial=0
  Define CM Dict3 : CarMaker4SL/Define CM Dict  xname=ESP.User.ABS_off  xmono=off  xtype=Char  xdvaplace=IO_Out  xnstates=2  xfirststate=0  xinitial=0
  Define CM Dict4 : CarMaker4SL/Define CM Dict  xname=ESP.User.ESP_all_off  xmono=off  xtype=Char  xdvaplace=IO_Out  xnstates=2  xfirststate=0  xinitial=0
  Define CM Dict5 : CarMaker4SL/Define CM Dict  xname=ESP.User.Drive  xmono=off  xtype=Char  xdvaplace=IO_Out  xnstates=3  xfirststate=1  xinitial=1
  Define CM Dict6 : CarMaker4SL/Define CM Dict  xname=ESP.User.SideSlip_estimator_on  xmono=off  xtype=Char  xdvaplace=IO_Out  xnstates=2  xfirststate=0  xinitial=0
  Define CM Dict7 : CarMaker4SL/Define CM Dict  xname=ESP.User.mue_estimator_on  xmono=off  xtype=Char  xdvaplace=IO_Out  xnstates=2  xfirststate=0  xinitial=0
  Define CM Dict8 : CarMaker4SL/Define CM Dict  xname=ESP.User.DiffLockDVA_on  xmono=off  xtype=Char  xdvaplace=IO_Out  xnstates=2  xfirststate=0  xinitial=0
  Define CM Dict9 : CarMaker4SL/Define CM Dict  xname=ESP.User.DiffLockDVA_Trq  xunit=Nm  xmono=off  xtype=Double4  xdvaplace=IO_Out  xnstates=2  xfirststate=0  xinitial=0
  Read CM Dict1 : CarMaker4SL/Read CM Dict  xname=ESP.User.Drive  xsync=off  xstime=Continuous
  Read CM Dict10 : CarMaker4SL/Read CM Dict  xname=ESP.User.HSA_off  xsync=off  xstime=Continuous
  Read CM Dict11 : CarMaker4SL/Read CM Dict  xname=ESP.User.oneWheel_on  xsync=off  xstime=Continuous
  Read CM Dict2 : CarMaker4SL/Read CM Dict  xname=ESP.User.ESP_all_off  xsync=off  xstime=Continuous
  Read CM Dict3 : CarMaker4SL/Read CM Dict  xname=ESP.User.ESP_off  xsync=off  xstime=Continuous
  Read CM Dict4 : CarMaker4SL/Read CM Dict  xname=ESP.User.ASR_off  xsync=off  xstime=Continuous
  Read CM Dict5 : CarMaker4SL/Read CM Dict  xname=ESP.User.ABS_off  xsync=off  xstime=Continuous
  Read CM Dict6 : CarMaker4SL/Read CM Dict  xname=ESP.User.SideSlip_estimator_on  xsync=off  xstime=Continuous
  Read CM Dict7 : CarMaker4SL/Read CM Dict  xname=ESP.User.mue_estimator_on  xsync=off  xstime=Continuous
  Read CM Dict8 : CarMaker4SL/Read CM Dict  xname=ESP.User.DiffLockDVA_on  xsync=off  xstime=Continuous
  Read CM Dict9 : CarMaker4SL/Read CM Dict  xname=ESP.User.DiffLockDVA_Trq  xsync=off  xstime=Continuous
  User_In : Outport  VectorParamsAs1DForOutWhenUnconnected=off
  wires:
  Read CM Dict1/1 -> Bus Creator1/1  "User_Drive"
  Bus Creator1/1 -> User_In/1
  Read CM Dict5/1 -> Bus Creator2/4  "User_Switch_ABS_off"
  Read CM Dict4/1 -> Bus Creator2/3  "User_Switch_ASR_off"
  Read CM Dict3/1 -> Bus Creator2/2  "User_Switch_ESP_off"
  Read CM Dict2/1 -> Bus Creator2/1  "User_Switch_Main_off"
  Bus Creator2/1 -> Bus Creator1/2  "User_Switch"
  Read CM Dict6/1 -> Bus Creator3/1  "User_SideSlip_estimator_on"
  Read CM Dict7/1 -> Bus Creator3/2  "User_mue_estimator_on"
  Bus Creator3/1 -> Bus Creator1/3  "User_estimators_on"
  Read CM Dict8/1 -> Bus Creator4/1  "User_DiffLock_on"
  Read CM Dict9/1 -> Bus Creator4/2  "User_DiffLock_Trq"
  Bus Creator4/1 -> Bus Creator1/4  "User_DiffLock"
  Read CM Dict10/1 -> Bus Creator2/5  "User_Switch_HSA_off"
  Read CM Dict11/1 -> Bus Creator1/5  "User_oneWheel_on"

== system generic_src/CarMaker/IPG Vehicle/Brake/HydBrakeCU Example/ESP Controller/Vehicle Input Parameter ==
  note: Note:
      | We could also use
      | the left wheel as is has
      | the same coordinate
      | as regards x-axis
      | (which interests us here)
  note: Note:
      | We could also use
      | the left wheel as is has
      | the same coordinate
      | as regards x-axis
      | (which interests us here)
  Bus Creator{,1..3} (4 alike) : BusCreator  Inputs=4
  Bus Creator4 : BusCreator  Inputs=2
  Read CM Parameter : CarMaker4SL/Read CM Parameter  xfile=TireFL  xkey=KinRollRadius  xnout=1  xdefaults=0  xmuxed=on  xstime=Continuous
      settings: SourceProductName=CarMaker4SL
  Read CM Parameter1 : CarMaker4SL/Read CM Parameter  xfile=TireFR  xkey=KinRollRadius  xnout=1  xdefaults=0  xmuxed=on  xstime=Continuous
      settings: SourceProductName=CarMaker4SL
  Read CM Parameter2 : CarMaker4SL/Read CM Parameter  xfile=TireRL  xkey=KinRollRadius  xnout=1  xdefaults=0  xmuxed=on  xstime=Continuous
      settings: SourceProductName=CarMaker4SL
  Read CM Parameter3 : CarMaker4SL/Read CM Parameter  xfile=TireRR  xkey=KinRollRadius  xnout=1  xdefaults=0  xmuxed=on  xstime=Continuous
      settings: SourceProductName=CarMaker4SL
  Read CM Parameter4 : CarMaker4SL/Read CM Parameter  xfile=Vehicle  xkey=WheelCarrier.fr.pos  xnout=1  xdefaults=0  xmuxed=on  xstime=Continuous
      settings: SourceProductName=CarMaker4SL
  Read CM Parameter5 : CarMaker4SL/Read CM Parameter  xfile=Vehicle  xkey=Body.pos  xnout=1  xdefaults=0  xmuxed=on  xstime=Continuous
      settings: SourceProductName=CarMaker4SL
  Read CM Parameter6 : CarMaker4SL/Read CM Parameter  xfile=Vehicle  xkey=Body.pos  xnout=1  xdefaults=0  xmuxed=on  xstime=Continuous
      settings: SourceProductName=CarMaker4SL
  Read CM Parameter7 : CarMaker4SL/Read CM Parameter  xfile=Vehicle  xkey=WheelCarrier.rr.pos  xnout=1  xdefaults=0  xmuxed=on  xstime=Continuous
      settings: SourceProductName=CarMaker4SL
  Read CM Parameter8 : CarMaker4SL/Read CM Parameter  xfile=Vehicle  xkey=WheelCarrier.rl.pos  xnout=2  xdefaults=0  xmuxed=off  xstime=Continuous
      settings: SourceProductName=CarMaker4SL
  Read CM Parameter9 : CarMaker4SL/Read CM Parameter  xfile=Vehicle  xkey=WheelCarrier.fl.pos  xnout=2  xdefaults=0  xmuxed=off  xstime=Continuous
      settings: SourceProductName=CarMaker4SL
  Steer Angle y-Data : Constant  Value=SteerAng_Out
  Steer Wheel Angle x-Data : Constant  Value=SteerWheelAng_In
  Sum3 : Sum  Inputs=+-  InputSameDT=on  SaturateOnIntegerOverflow=on  OutDataTypeStr=Inherit: Same as first input
  Sum4 : Sum  Inputs=+-  InputSameDT=on  SaturateOnIntegerOverflow=on  OutDataTypeStr=Inherit: Same as first input
  Terminator{,1..9} (10 alike) : Terminator
  z-Position of WheelCarrier FL : CarMaker4SL/Read CM Parameter  xfile=Vehicle  xkey=WheelCarrier.fl.pos  xnout=3  xdefaults=0  xmuxed=off  xstime=Continuous
      settings: SourceProductName=CarMaker4SL
  z-Position of WheelCarrier FR : CarMaker4SL/Read CM Parameter  xfile=Vehicle  xkey=WheelCarrier.fr.pos  xnout=3  xdefaults=0  xmuxed=off  xstime=Continuous
      settings: SourceProductName=CarMaker4SL
  z-Position of WheelCarrier RL : CarMaker4SL/Read CM Parameter  xfile=Vehicle  xkey=WheelCarrier.rl.pos  xnout=3  xdefaults=0  xmuxed=off  xstime=Continuous
      settings: SourceProductName=CarMaker4SL
  z-Position of WheelCarrier RR : CarMaker4SL/Read CM Parameter  xfile=Vehicle  xkey=WheelCarrier.rr.pos  xnout=3  xdefaults=0  xmuxed=off  xstime=Continuous
      settings: SourceProductName=CarMaker4SL
  Vehicle Param : Outport  VectorParamsAs1DForOutWhenUnconnected=off
  wires:
  Bus Creator1/1 -> Vehicle Param/1
  Read CM Parameter1/1 -> Bus Creator/2  "Param_RadiusFR"
  Read CM Parameter3/1 -> Bus Creator/4  "Param_RadiusRR"
  Bus Creator/1 -> Bus Creator1/1  "TireRadius"
  Read CM Parameter/1 -> Bus Creator/1  "Param_RadiusFL"
  Read CM Parameter2/1 -> Bus Creator/3  "Param_RadiusRL"
  Read CM Parameter5/1 -> Sum4/2
  Read CM Parameter4/1 -> Sum4/1
  Sum4/1 -> Bus Creator2/1  "Param_aF"
  Read CM Parameter7/1 -> Sum3/2
  Sum3/1 -> Bus Creator2/2  "Param_aR"
  Read CM Parameter6/1 -> Sum3/1
  Bus Creator2/1 -> Bus Creator1/2  "VehicleGeometry"
  Read CM Parameter8/2 -> Bus Creator2/4  "Param_bR"
  Read CM Parameter9/2 -> Bus Creator2/3  "Param_bF"
  Read CM Parameter9/1 -> Terminator/1
  Read CM Parameter8/1 -> Terminator1/1
  z-Position of WheelCarrier FL/1 -> Terminator2/1
  z-Position of WheelCarrier FL/2 -> Terminator3/1
  Bus Creator3/1 -> Bus Creator1/3  "CarrierGeometry"
  z-Position of WheelCarrier FL/3 -> Bus Creator3/1  "Param_zFL"
  z-Position of WheelCarrier FR/3 -> Bus Creator3/2  "Param_zFR"
  z-Position of WheelCarrier RL/3 -> Bus Creator3/3  "Param_zRL"
  z-Position of WheelCarrier RR/3 -> Bus Creator3/4  "Param_zRR"
  z-Position of WheelCarrier FR/1 -> Terminator4/1
  z-Position of WheelCarrier FR/2 -> Terminator5/1
  z-Position of WheelCarrier RL/1 -> Terminator6/1
  z-Position of WheelCarrier RL/2 -> Terminator7/1
  z-Position of WheelCarrier RR/1 -> Terminator8/1
  z-Position of WheelCarrier RR/2 -> Terminator9/1
  Steer Angle y-Data/1 -> Bus Creator4/2  "SteerAng_Out"
  Steer Wheel Angle x-Data/1 -> Bus Creator4/1  "SteerWheelAng_In"
  Bus Creator4/1 -> Bus Creator1/4  "SteeringGeometry"

== system generic_src/CarMaker/IPG Vehicle/Brake/HydBrakeCU Example/HydBrakeCtrl_In/CreateBus HydBrakeCU ==
  In : Inport
  BusCreator : BusCreator  Inputs=45
  Demux : Demux  Outputs=45
      settings: DisplayOption=none
  Ground{,1..14} (15 alike) : Ground
  Terminator{,1..14} (15 alike) : Terminator
  Out : Outport  VectorParamsAs1DForOutWhenUnconnected=off
  wires:
  In/1 -> Demux/1
  BusCreator/1 -> Out/1
  Demux/1 -> BusCreator/1  "HydBrakeCU Pedal"
  Demux/2 -> BusCreator/2  "HydBrakeCU Park"
  Demux/3 -> BusCreator/3  "HydBrakeCU Trq_BrakeReg_max_FL"
  Demux/4 -> BusCreator/4  "HydBrakeCU Trq_BrakeReg_max_FR"
  Demux/5 -> BusCreator/5  "HydBrakeCU Trq_BrakeReg_max_RL"
  Demux/6 -> BusCreator/6  "HydBrakeCU Trq_BrakeReg_max_RR"
  Demux/7 -> BusCreator/7  "HydBrakeCU Trq_BrakeReg_FL"
  Demux/8 -> BusCreator/8  "HydBrakeCU Trq_BrakeReg_FR"
  Demux/9 -> BusCreator/9  "HydBrakeCU Trq_BrakeReg_RL"
  Demux/10 -> BusCreator/10  "HydBrakeCU Trq_BrakeReg_RR"
  Demux/11 -> BusCreator/11  "HydBrakeCU T_env"
  Demux/12 -> BusCreator/12  "HydBrakeCU Trq_WB_FL"
  Demux/13 -> BusCreator/13  "HydBrakeCU Trq_WB_FR"
  Demux/14 -> BusCreator/14  "HydBrakeCU Trq_WB_RL"
  Demux/15 -> BusCreator/15  "HydBrakeCU Trq_WB_RR"
  Demux/16 -> BusCreator/16  "HydBrakeCU Trq_PB_FL"
  Demux/17 -> BusCreator/17  "HydBrakeCU Trq_PB_FR"
  Demux/18 -> BusCreator/18  "HydBrakeCU Trq_PB_RL"
  Demux/19 -> BusCreator/19  "HydBrakeCU Trq_PB_RR"
  Demux/20 -> BusCreator/20  "HydBrakeCU Rel_SW"
  Demux/21 -> BusCreator/21  "HydBrakeCU pMC"
  Demux/22 -> BusCreator/22
  Demux/23 -> Terminator14/1  "HydBrakeCU pWB_FL"
  Demux/24 -> BusCreator/24  "HydBrakeCU pWB_FR"
  Demux/25 -> BusCreator/25  "HydBrakeCU pWB_RL"
  Demux/26 -> BusCreator/26  "HydBrakeCU pWB_RR"
  Demux/27 -> BusCreator/27  "HydBrakeCU PuRetVolt"
  Demux/28 -> BusCreator/28  "HydBrakeCU PedFrc"
  Demux/29 -> BusCreator/29  "HydBrakeCU PedTravel"
  Demux/30 -> BusCreator/30  "HydBrakeCU PistTravel"
  Demux/45 -> Terminator/1
  Demux/44 -> Terminator1/1
  Demux/43 -> Terminator2/1
  Demux/42 -> Terminator3/1
  Demux/41 -> Terminator4/1
  Demux/40 -> Terminator5/1
  Demux/39 -> Terminator6/1
  Demux/38 -> Terminator7/1
  Demux/37 -> Terminator8/1
  Demux/36 -> Terminator9/1
  Demux/35 -> Terminator10/1
  Demux/34 -> Terminator11/1
  Demux/33 -> Terminator12/1
  Demux/32 -> Terminator13/1
  Ground/1 -> BusCreator/45
  Ground1/1 -> BusCreator/44
  Ground2/1 -> BusCreator/43
  Ground3/1 -> BusCreator/42
  Ground4/1 -> BusCreator/41
  Ground5/1 -> BusCreator/40
  Ground6/1 -> BusCreator/39
  Ground7/1 -> BusCreator/38
  Ground8/1 -> BusCreator/37
  Ground9/1 -> BusCreator/36
  Ground10/1 -> BusCreator/35
  Ground11/1 -> BusCreator/34
  Ground12/1 -> BusCreator/33
  Ground13/1 -> BusCreator/32
  Demux/31 -> BusCreator/31  "HydBrakeCU DiaphTravel"
  Ground14/1 -> BusCreator/23

== system generic_src/CarMaker/IPG Vehicle/Brake/HydBrakeCU Example/HydBrakeCtrl_In/CreateBus HydBrakeCU_Cfg ==
  In : Inport
  BusCreator : BusCreator  Inputs=4
  Demux : Demux
      settings: DisplayOption=none
  Ground : Ground
  Terminator : Terminator
  Out : Outport  VectorParamsAs1DForOutWhenUnconnected=off
  wires:
  In/1 -> Demux/1
  BusCreator/1 -> Out/1
  Demux/1 -> BusCreator/1  "HydBrakeCU_Cfg VhclClassId"
  Demux/2 -> BusCreator/2  "HydBrakeCU_Cfg nWheels"
  Demux/3 -> BusCreator/3  "HydBrakeCU_Cfg BrakeKind"
  Ground/1 -> BusCreator/4
  Demux/4 -> Terminator/1

== system generic_src/CarMaker/IPG Vehicle/CarAndTrailer/Forces/Suspension Forces/Suspension External Forces Update ==
  Bus Creator21 : BusCreator  Inputs=6
  Bus Creator22 : BusCreator  Inputs=4
  Bus Creator23 : BusCreator  Inputs=4
  Ground{32..39} (8 alike) : Ground
  Out1 : Outport
  wires:
  Ground37/1 -> Bus Creator22/2
  Ground38/1 -> Bus Creator22/3
  Ground39/1 -> Bus Creator22/4
  Ground35/1 -> Bus Creator23/4
  Bus Creator21/1 -> Out1/1
  Bus Creator22/1 -> Bus Creator21/6
  Ground33/1 -> Bus Creator23/2
  Bus Creator23/1 -> Bus Creator21/5
  [C] -> Bus Creator21/3
  Ground32/1 -> Bus Creator23/1
  Ground34/1 -> Bus Creator23/3
  [B] -> Bus Creator21/2
  [A] -> Bus Creator21/1
  Ground36/1 -> Bus Creator22/1
  [D] -> Bus Creator21/4

== system generic_src/CarMaker/IPG Vehicle/CarAndTrailer/Forces/Tires/TireFL ==
  note: Insert your tire model here.
  Sync_In : Inport
  Load : Inport  Port=2
  vxtrans : Inport  Port=3
  vytrans : Inport  Port=4
  Rim_rotv : Inport  Port=5
  Rim_turnv : Inport  Port=6
  InclinAngle : Inport  Port=7
  muRoad : Inport  Port=8
  Ground{1..11} (11 alike) : Ground
  Terminator{,1..6,12} (8 alike) : Terminator
  Slp : Outport  VectorParamsAs1DForOutWhenUnconnected=off
  Alpha : Outport  Port=2  VectorParamsAs1DForOutWhenUnconnected=off
  TurnSlp : Outport  Port=3  VectorParamsAs1DForOutWhenUnconnected=off
  rBelt_eff : Outport  Port=4  VectorParamsAs1DForOutWhenUnconnected=off
  vBelt : Outport  Port=5  VectorParamsAs1DForOutWhenUnconnected=off
  LongFrc : Outport  Port=6  VectorParamsAs1DForOutWhenUnconnected=off
  SideFrc : Outport  Port=7  VectorParamsAs1DForOutWhenUnconnected=off
  LoadFrc : Outport  Port=8  VectorParamsAs1DForOutWhenUnconnected=off
  OverturnTrq : Outport  Port=9  VectorParamsAs1DForOutWhenUnconnected=off
  RollResist : Outport  Port=10  VectorParamsAs1DForOutWhenUnconnected=off
  AlignTrq : Outport  Port=11  VectorParamsAs1DForOutWhenUnconnected=off
  wires:
  Ground11/1 -> vBelt/1
  Ground10/1 -> rBelt_eff/1
  Ground9/1 -> TurnSlp/1
  Rim_turnv/1 -> Terminator6/1
  Sync_In/1 -> Terminator12/1
  Ground2/1 -> Alpha/1
  Ground3/1 -> LongFrc/1
  Ground4/1 -> SideFrc/1
  Ground5/1 -> OverturnTrq/1
  vxtrans/1 -> Terminator1/1
  vytrans/1 -> Terminator2/1
  Rim_rotv/1 -> Terminator3/1
  InclinAngle/1 -> Terminator4/1
  muRoad/1 -> Terminator5/1
  Load/1 -> Terminator/1
  Ground1/1 -> Slp/1
  Ground6/1 -> LoadFrc/1
  Ground7/1 -> RollResist/1
  Ground8/1 -> AlignTrq/1
